simulink model "ev_fuzzy"  (R2025a)
settings: Solver=ode3  StartTime=0.0  StopTime=10.0  FixedStep=1e-4  RelTol=1e-3
libraries: fl_lib x5, nesl_utility x4, simulink x2, fuzblock x1, spsPVArrayLib x1, sps_lib x1
settings Model: Creator=kedha  LastModifiedBy=Rishitha

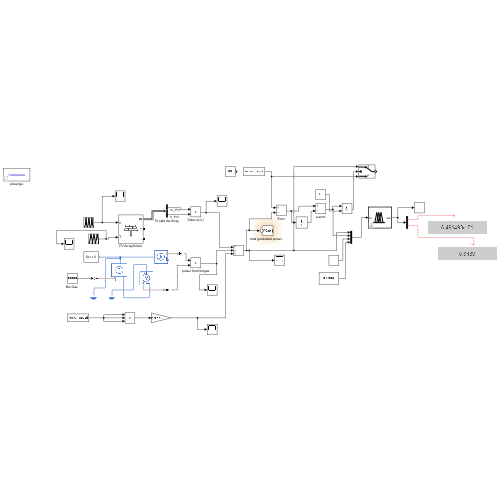
[thumbnail: Simulink's stored preview of the top-level diagram]
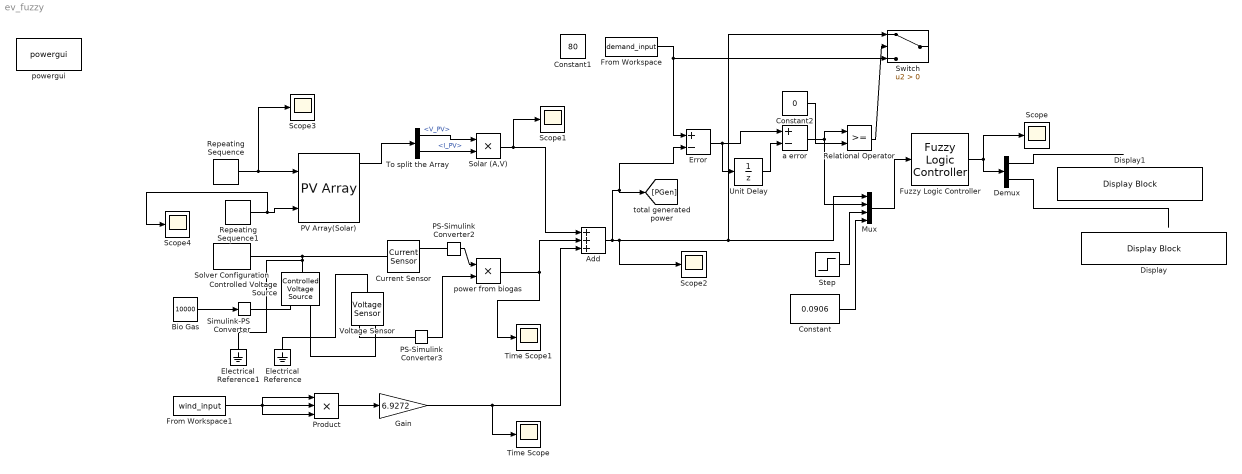
== system ev_fuzzy ==
  Add : Sum  Inputs=+++
  "Bio Gas " : Constant  Value=10000
  Constant : Constant  Value=0.0906
  Constant1 : Constant  Value=80
  Constant2 : Constant  Value=0
  Controlled Voltage Source : fl_lib/Electrical/Electrical Sources/Controlled Voltage Source
  Current Sensor : fl_lib/Electrical/Electrical Sensors/Current Sensor
  Demux : Demux  Outputs=2
  Display : DisplayBlock  LabelPosition=Hide  Transparency=1  GridColor=[0.502, 0.502, 0.502]
  Display1 : DisplayBlock  LabelPosition=Hide  Format=Custom  Transparency=1  GridColor=[0.502, 0.502, 0.502]
  Electrical Reference : fl_lib/Electrical/Electrical Elements/Electrical Reference
  Electrical Reference1 : fl_lib/Electrical/Electrical Elements/Electrical Reference
  Error : Sum  Inputs=+-
  From Workspace : FromWorkspace  VariableName=demand_input
  From Workspace1 : FromWorkspace  VariableName=wind_input
  Fuzzy Logic Controller : fuzblock/Fuzzy Logic  Controller  FIS="\"C:\\SEM-5\\Control Systems\\Project\\evcs_fuzzy.fis\""  OutputSampleNumber=101  DataType=double  UseLookupTable=on  NumBreakpoints=4  FuzzifiedInputs=off  RuleFiringStrengths=off  RuleOutputs=off  AggregatedOutputs=off  SimulateUsing=Interpreted execution  OutOfRangeInputValueMessage=warning  NoRuleFiredMessage=warning  EmptyOutputFuzzySetMessage=warning
  Gain : Gain  Gain=6.9272
  Mux : Mux
  PS-Simulink Converter2 : nesl_utility/PS-Simulink Converter  PhysicalDomain=network_engine_domain  SubClassName=ps_output  LeftPortType=input  RightPortType=output  PseudoPeriodic=off  Frequencies=[]  VectorFormat=inherit  Unit=inherit  AffineConversion=off
  PS-Simulink Converter3 : nesl_utility/PS-Simulink Converter  PhysicalDomain=network_engine_domain  SubClassName=ps_output  LeftPortType=input  RightPortType=output  PseudoPeriodic=off  Frequencies=[]  VectorFormat=inherit  Unit=inherit  AffineConversion=off
  PV Array(Solar) : spsPVArrayLib/PV Array  Npar=4  Nser=10  PlotType=array @ 1000 W/m2 & specified temperatures  S_vec="[ 1000  500  100 ]"  Temp_C_vec="[ 45 25  ]"  ModuleName=Trina Solar TSM-275PA14  PlotWhenSelected=off  Pm=275.328  Ncell=72  Voc=44.4  Isc=8.39  Vm=35.85  Im=7.68  beta_Voc_pc=-0.36  alpha_Isc_pc=0.06  beta_Voc=-0.15984  alpha_Isc=0.005034  IL=8.4178  I0=2.8124e-10  nI=0.99686  Rsh=121.4327  Rs=0.40249  RobustModel=off  RobustCellTemperature=313.3991  BAL=on  Tc=1e-6  Tfilter=5e-5
  Product : Product  Inputs=3
  Relational Operator : RelationalOperator  OutDataTypeStr=boolean  RndMeth=Simplest  InputSameDT=off
  Repeating Sequence : simulink/Sources/Repeating Sequence  rep_seq_t=[0 7 12 17 24]  rep_seq_y=[0 200 1000 200 0]
  Repeating Sequence1 : simulink/Sources/Repeating Sequence  rep_seq_t=[0 7 14 24]  rep_seq_y=[20 25 35 25]
  Scope{,1..4} (5 alike) : Scope
      Scope settings: ActiveDisplayYMinimum=0.45444881889763783  ActiveDisplayYMaximum=0.9099606299212597
      Scope1 settings: ActiveDisplayYMinimum=-1  ActiveDisplayYMaximum=1
      Scope2 settings: ActiveDisplayYMinimum=11419.992288603986  ActiveDisplayYMaximum=16922.085402564142  DataLoggingVariableName=ScopeData2
      Scope3 settings: DataLoggingVariableName=ScopeData5
      Scope4 settings: DataLoggingVariableName=ScopeData6
  Simulink-PS Converter : nesl_utility/Simulink-PS Converter  PhysicalDomain=network_engine_domain  SubClassName=ps_input  LeftPortType=input  RightPortType=output  PseudoPeriodic=off  Frequencies=[]  NoiseDistribution=none  NoiseParameters=[]  Unit=1  AffineConversion=off  FilteringAndDerivatives=provide  SimscapeFilterOrder=1  InputFilterTimeConstant=0.001  UdotUserProvided=0
  Solar (A,V) : Product
  Solver Configuration : nesl_utility/Solver Configuration  PhysicalDomain=network_engine_domain  SubClassName=solver  LeftPortType=input  RightPortType=generic  Tones=[]  Harmonics=[]  SimulateNoise=off  Profile=off  UseLocalSampling=off  EnableSwitchedLinearOptims=on  FrequencyDomain=off  UseCCode=off  RelTol=0.001  AbsTol=0.001  MinStep=1e-09  ToWorkspace=off  RevertToSquareIcSolve=off  NumHomotopyIterations=100  PhasorMode=off  PhasorModeNumHarmonics=1  ConsistencySolver=NEWTON_XTOL_AFTER_FTOL  IndexReductionMethod=DerivativeReplacement  DoDC=off  ResidualTolerance=1e-09  ConsistencyTolSource=GLOBAL  ConsistencyAbsTol=0.001  ConsistencyRelTol=0.001  ConsistencyTolFactor=0.001  UseLocalSolver=off  LocalSolverChoice=NE_BACKWARD_EULER_ADVANCER  ResolveIndetEquations=on  FunctionEvalNumThread=1  LocalSolverSampleTime=0.001  DoFixedCost=off  MaxNonlinIter=3  MaxModeIter=2  ComputeImpulses=off  ImpulseIterations=2  LinearAlgebra=auto  LinearAlgebraNumThread=0  EquationFormulation=NE_TIME_EF  DelaysMemoryBudget=1024  AutomaticFiltering=on  FilteringTimeConstant=0.001  PartitionStorageMethod=AS_NEEDED  PartitionMemoryBudget=1024  PartitionMethod=ROBUST  MultibodyUseLocalSolver=off  MultibodyLocalSolverChoice=ODE1  MultibodyLocalSolverSampleTime=0.001
  Step : Step  Time=17  SampleTime=0
  Switch : Switch  Criteria=u2 > Threshold  SaturateOnIntegerOverflow=off  InputSameDT=off
  Time Scope : Scope
      settings: TimeUnits=Metric (based on Time Span)  ActiveDisplayYMinimum=8056.6233100791951  ActiveDisplayYMaximum=22006.056566399078  YLabel=Amplitude  DataLoggingVariableName=ScopeData3
  Time Scope1 : Scope
      settings: TimeUnits=Metric (based on Time Span)  ActiveDisplayYMinimum=-1  ActiveDisplayYMaximum=1  YLabel=Amplitude  DataLoggingVariableName=ScopeData4
  To split the Array : BusSelector  OutputSignals=V_PV,I_PV
  Unit Delay : UnitDelay  SampleTime=-1  HasFrameUpgradeWarning=on
  Voltage Sensor : fl_lib/Electrical/Electrical Sensors/Voltage Sensor
  a error : Sum  Inputs=+-
  power from biogas : Product
  powergui : sps_lib/powergui  Priority=1  SimulationMode=Continuous  SampleTime=50e-6  frequency=60  Iterations=50  frequencyindice=0  Pbase=100e6  ErrMax=1e-4  UnitsV=kV  UnitsW=MW  buscounter=0  FunctionMessages=off  echomessages=off  EnableUseOfTLC=off  CurrentSourceSwitches=off  DisableSnubberDevices=off  DisableRonSwitches=off  DisableVfSwitches=off  DisplayEquations=off  AutomaticDiscreteSolvers=off  SolverType=Tustin/Backward Euler (TBE)  Interpol=off  ExternalGateDelay=off  methode=off  Ts=100  x0status=blocks  SPID=on  SwTol=0  HookPort=off  NonlinearTolerance=1e-4  nMaxIteration=100  ContinueOnMaxIteration=off  RestoreLinks=warning  ResistiveCurrentMeasurement=off  Frange=[0:2:500]  Ylog=off  Xlog=on  ShowGrid=off  save=off  variable=ZData  structure=0  ZoomFFT=off  StartTime=0.0  cycles=1  DisplayStyle=1  fundamental=60  FreqAxis=off  MaxFrequency=1000  frequencyindicesteady=1  RmsSteady=1  display=off
  wires:
  PV Array(Solar)/1 -> To split the Array/1
  To split the Array/1 -> Solar (A,V)/1  "<V_PV>"
  To split the Array/2 -> Solar (A,V)/2  "<I_PV>"
  Solar (A,V)/1 -> Scope1/1, Add/1
  Repeating Sequence/1 -> Scope3/1, PV Array(Solar)/1
  "Bio Gas "/1 -> Simulink-PS Converter/1
  PS-Simulink Converter3/1 -> power from biogas/2
  PS-Simulink Converter2/1 -> power from biogas/1
  power from biogas/1 -> Time Scope1/1, Add/2
  Error/1 -> a error/1, Unit Delay/1
  Unit Delay/1 -> a error/2
  From Workspace1/1 -> Product/3, Product/2, Product/1
  Product/1 -> Gain/1
  Gain/1 -> Time Scope/1, Add/3
  Add/1 -> Switch/1, Mux/1, Scope2/1, Error/2, [PGen]
  Step/1 -> Mux/3
  Constant/1 -> Mux/4
  Mux/1 -> Fuzzy Logic Controller/1
  Fuzzy Logic Controller/1 -> Scope/1, Demux/1
  Demux/1 -> ?
  Demux/2 -> ?
  Relational Operator/1 -> Switch/2
  Repeating Sequence1/1 -> Scope4/1, PV Array(Solar)/2
  From Workspace/1 -> Switch/3, Error/1
  a error/1 -> Mux/2, Relational Operator/1
  Constant2/1 -> Relational Operator/2
  connections:
  Simulink-PS Converter/RConn1 -- Controlled Voltage Source/RConn1
  Controlled Voltage Source/LConn1 -- Electrical Reference1/LConn1 -- Solver Configuration/RConn1 -- Current Sensor/LConn1
  Controlled Voltage Source/RConn2 -- Voltage Sensor/RConn2
  Voltage Sensor/RConn1 -- PS-Simulink Converter3/LConn1
  Current Sensor/RConn1 -- PS-Simulink Converter2/LConn1
  Voltage Sensor/LConn1 -- Electrical Reference/LConn1
